simulink model "L2_scheme"  (R2025b)
settings: Solver=VariableStepAuto  StartTime=0.0  StopTime=10.0  RelTol=1e-3
settings Model: Creator=yzhar  LastModifiedBy=yzhar

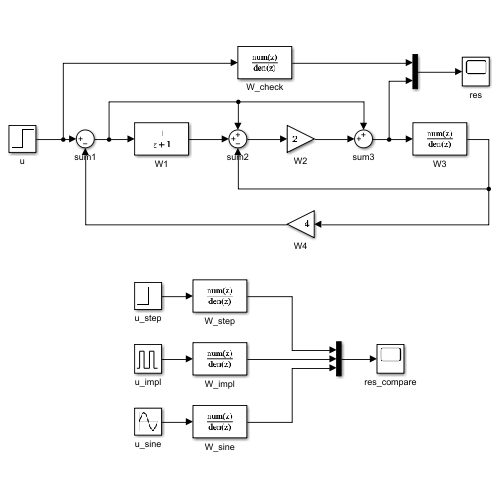
[thumbnail: Simulink's stored preview of the top-level diagram]
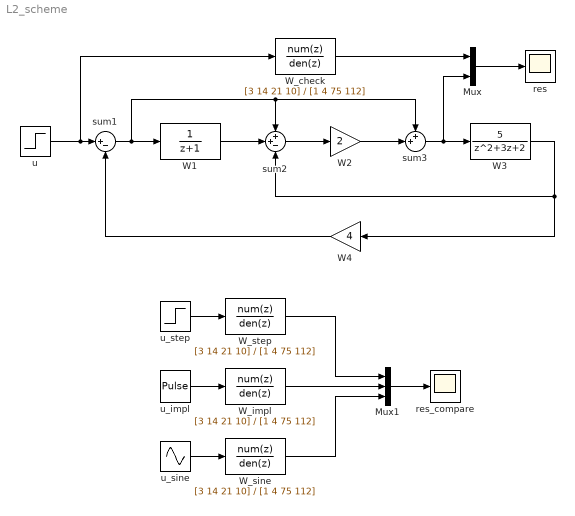
== system L2_scheme ==
  Mux : Mux  Inputs=2
  Mux1 : Mux  Inputs=3
  W1 : DiscreteTransferFcn  Denominator=[1 1]
  W2 : Gain  Gain=2
  W3 : DiscreteTransferFcn  Numerator=[5]  Denominator=[1 3 2]
  W4 : Gain  Gain=4
  W_check : DiscreteTransferFcn  Numerator=[3 14 21 10]  Denominator=[1 4 75 112]
  W_impl : DiscreteTransferFcn  Numerator=[3 14 21 10]  Denominator=[1 4 75 112]
  W_sine : DiscreteTransferFcn  Numerator=[3 14 21 10]  Denominator=[1 4 75 112]
  W_step : DiscreteTransferFcn  Numerator=[3 14 21 10]  Denominator=[1 4 75 112]
  res : Scope
      settings: ActiveDisplayYMinimum=-1.2863751525491946E+42  ActiveDisplayYMaximum=3.6595201315527205E+42
  res_compare : Scope
      settings: ActiveDisplayYMinimum=-3.1287221730350781E+44  ActiveDisplayYMaximum=5.9854271295530761E+44
  sum1 : Sum  Inputs=|+-
  sum2 : Sum  Inputs=++-
  sum3 : Sum  Inputs=++|
  u : Step  SampleTime=0
  u_impl : DiscretePulseGenerator  PulseType=Time based  Period=10  PulseWidth=5
  u_sine : Sin  SampleTime=0
  u_step : Step  SampleTime=0
  wires:
  u/1 -> W_check/1, sum1/1
  sum1/1 -> sum3/1, sum2/1, W1/1
  W1/1 -> sum2/2
  sum2/1 -> W2/1
  W2/1 -> sum3/2
  sum3/1 -> Mux/2, W3/1
  W3/1 -> W4/1, sum2/3
  W4/1 -> sum1/2
  W_check/1 -> Mux/1
  Mux/1 -> res/1
  W_impl/1 -> Mux1/2
  W_step/1 -> Mux1/1
  W_sine/1 -> Mux1/3
  u_sine/1 -> W_sine/1
  u_impl/1 -> W_impl/1
  u_step/1 -> W_step/1
  Mux1/1 -> res_compare/1
